simulink model "induction_motor_load_step"  (R2021a)
settings: Solver=VariableStepAuto  StartTime=0.0  StopTime=3  FixedStep=0.000001  MaxStep=0.000001  MinStep=0.0000001  RelTol=1e-7
values from neighbouring files (symbols this model uses):
  A1 = [-1/(ts*sig) 0 lm/(ls*tr*sig) 0;0 -1/(ts*sig) 0 lm/(ls*tr*sig);lm/(lr*ts*sig) 0 -1/(tr*sig) 0; 0 lm/(lr*ts*sig) 0 -1/(tr*sig)]    [induction_motor_parameters.m]
  A2 = [0 1 0 0; -1 0 0 0;0 0 0 1;0 0 -1 0]    [induction_motor_parameters.m]
  A3 = [0 1/sig 0 lm/(ls*sig);-1/sig 0 -lm/(ls*sig) 0;0 -lm/(lr*sig) 0 -lm*lm/(ls*lr*sig); lm/(lr*sig) 0 lm*lm/(ls*lr*sig) 0]    [induction_motor_parameters.m]
  B = [1/(ls*sig) 0 0 0;0 1/(ls*sig) 0 0; -lm/(ls*lr*sig) 0 0 0;0 -lm/(ls*lr*sig) 0 0 ]    [induction_motor_parameters.m]
  fr = 0.0015    [induction_motor_parameters.m]
  j = 0.0056    [induction_motor_parameters.m]
  L = [ls 0 lm 0;0 ls 0 lm;lm 0 lr 0;0 lm 0 lr]    [induction_motor_parameters.m]
  lm = 0.069    [induction_motor_parameters.m]
  lr = 0.071    [induction_motor_parameters.m]
  p = 2    [induction_motor_parameters.m]
  T = [2/3 -1/3 -1/3 ; -1/3 2/3 -1/3;-1/3 -1/3 2/3]    [induction_motor_parameters.m]
  T_dent = t/m    (= 0.000952380952381)    [induction_motor_parameters.m]
libraries: spsabctodq0Lib x1, spsdq0toabcLib x1, simulink x1, spspowerguiLib x1

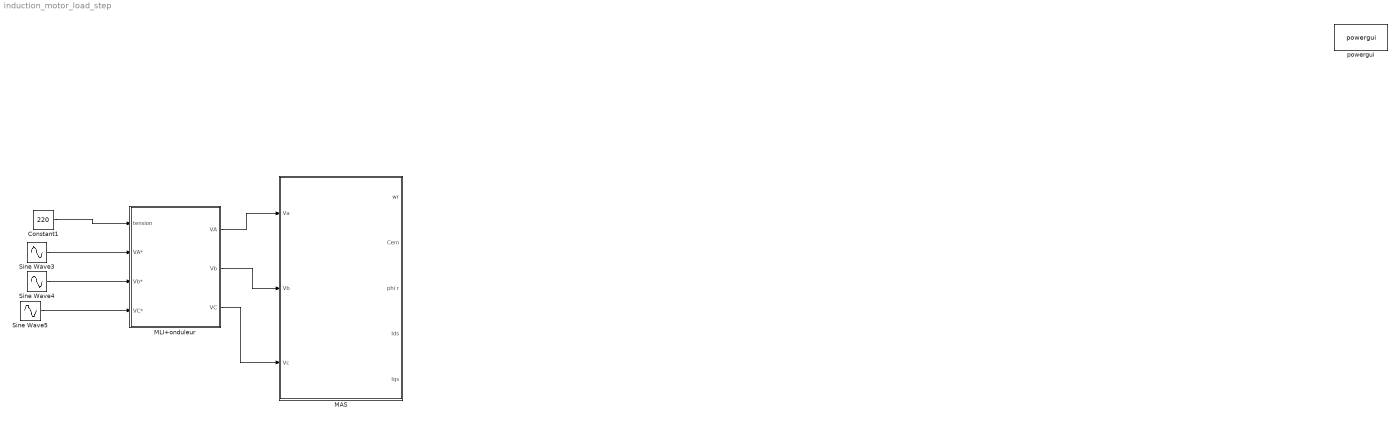
== system induction_motor_load_step ==
  Constant1 : Constant  Value=220
  "MAS " : Subsystem
  MLI+onduleur : Subsystem
  Sine Wave3 : Sin  Amplitude=220  Frequency=2*pi*50  SampleTime=0
  Sine Wave4 : Sin  Amplitude=220  Frequency=2*pi*50  Phase=-2*pi/3  SampleTime=0
  Sine Wave5 : Sin  Amplitude=220  Frequency=2*pi*50  Phase=-4*pi/3  SampleTime=0
  powergui : spspowerguiLib/powergui  Priority=1  SimulationMode=Discrete  SampleTime=50e-7  frequency=60  Iterations=50  frequencyindice=0  Pbase=100e6  ErrMax=1e-4  UnitsV=kV  UnitsW=MW  buscounter=0  FunctionMessages=off  echomessages=off  EnableUseOfTLC=off  CurrentSourceSwitches=off  DisableSnubberDevices=off  DisableRonSwitches=off  DisableVfSwitches=off  DisplayEquations=off  AutomaticDiscreteSolvers=off  SolverType=Tustin/Backward Euler (TBE)  Interpol=off  ExternalGateDelay=off  methode=off  Ts=100  x0status=blocks  SPID=on  SwTol=0  HookPort=off  NonlinearTolerance=1e-4  nMaxIteration=100  ContinueOnMaxIteration=off  RestoreLinks=warning  ResistiveCurrentMeasurement=off  Frange=[0:2:500]  Ylog=off  Xlog=on  ShowGrid=off  save=off  variable=ZData  structure=0  ZoomFFT=off  StartTime=0.0  cycles=1  DisplayStyle=1  fundamental=60  FreqAxis=off  MaxFrequency=1000  frequencyindicesteady=1  RmsSteady=1  display=off
  wires:
  MLI+onduleur/2(Vb) -> "MAS "/2(Vb)
  MLI+onduleur/3(VC) -> "MAS "/3(Vc)
  MLI+onduleur/1(VA) -> "MAS "/1(Va)
  Sine Wave3/1 -> MLI+onduleur/2(VA*)
  Sine Wave5/1 -> MLI+onduleur/4(VC*)
  Sine Wave4/1 -> MLI+onduleur/3(Vb*)
  Constant1/1 -> MLI+onduleur/1(tension)

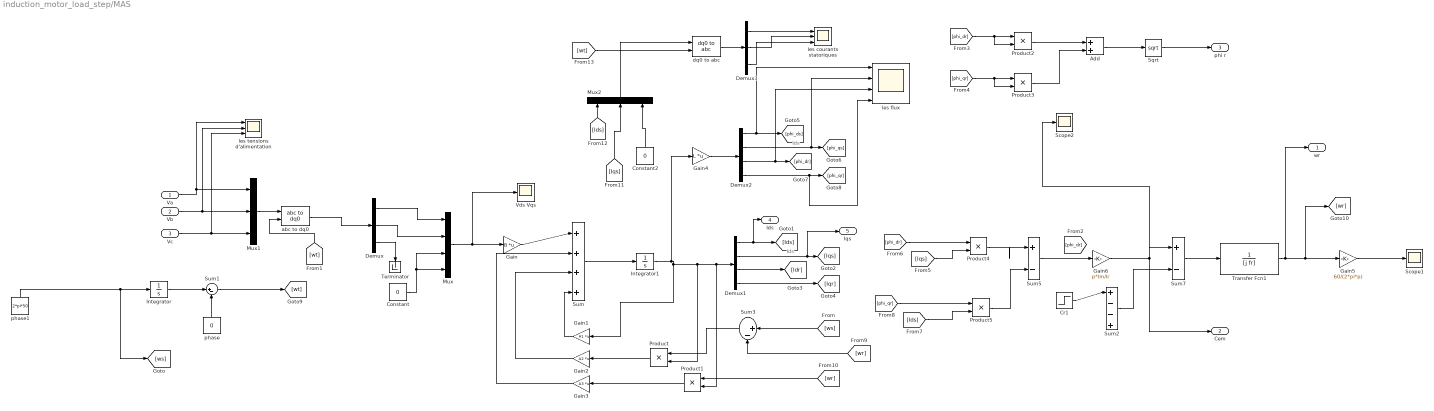
== system induction_motor_load_step/MAS  ==
  note: Ids
  note: Ids
  Va : Inport
  Vb : Inport  Port=2
  Vc : Inport  Port=3
  Add : Sum
  Constant : Constant  Value=0
  Constant2 : Constant  Value=0
  Cr1 : Step  After=10  SampleTime=0
  Demux : Demux  Outputs=3
  Demux1 : Demux
  Demux2 : Demux
  Demux3 : Demux  Outputs=3
  Gain : Gain  Gain=B  Multiplication=Matrix(K*u)
  Gain1 : Gain  Gain=A1  Multiplication=Matrix(K*u)
  Gain2 : Gain  Gain=A2  Multiplication=Matrix(K*u)
  Gain3 : Gain  Gain=A3  Multiplication=Matrix(K*u)
  Gain4 : Gain  Gain=L  Multiplication=Matrix(K*u)
  Gain5 : Gain  Gain=60/(2*pi*p)
  Gain6 : Gain  Gain=p*lm/lr
  Integrator : Integrator
  Integrator1 : Integrator
  Mux : Mux
  Mux1 : Mux  Inputs=3
  Mux2 : Mux  Inputs=3
  Product{,1..5} (6 alike) : Product
  Scope1 : Scope
  Scope2 : Scope
  Sqrt : Sqrt  SaturateOnIntegerOverflow=on
  Sum : Sum  Inputs=|++++
  Sum{1,3,5,7} (4 alike) : Sum  Inputs=|+-
  Sum2 : Sum  Inputs=|+--+
  Terminator : Terminator
  Transfer Fcn1 : TransferFcn  Denominator=[j fr]
  Vds Vqs : Scope
  abc to dq0 : spsabctodq0Lib/abc to dq0  Alignment=Aligned with phase A axis
  dq0 to abc : spsdq0toabcLib/dq0 to abc  Alignment=90 degrees behind phase A axis
  les courants statoriques : Scope  NumInputPorts=3
  les flux : Scope  NumInputPorts=4
  "les tensions d'alimentation " : Scope  NumInputPorts=3
  phase : Constant  Value=0
  phase1 : Constant  Value=2*pi*50
  wr : Outport
  Cem : Outport  Port=2
  phi r : Outport  Port=3
  Ids : Outport  Port=4
  Iqs : Outport  Port=5
  wires:
  Product/1 -> Gain2/1
  [wr] -> Product1/1
  Transfer Fcn1/1 -> wr/1, Gain5/1, [wr]
  Demux2/1 -> les flux/1, [phi_ds]
  Gain2/1 -> Sum/3
  Gain/1 -> Sum/1
  Constant2/1 -> Mux2/3
  Sum3/1 -> Product/1
  [Iqs] -> Product4/2
  Gain4/1 -> Demux2/1
  Demux2/3 -> les flux/3, [phi_dr]
  [wt] -> dq0 to abc/2
  Constant/1 -> Mux/4, Mux/3
  [phi_dr] -> Product4/1
  phase/1 -> Sum1/2
  Integrator1/1 -> Gain4/1, Product/2, Product1/2, Demux1/1, Gain1/1
  Demux/3 -> Terminator/1
  Demux/2 -> Mux/2
  [ws] -> Sum3/1
  Demux2/2 -> les flux/2, [phi_qs]
  Integrator/1 -> Sum1/1
  Demux1/4 -> [Iqr]
  Demux1/3 -> [Idr]
  Demux1/1 -> Ids/1, [Ids]
  Sum1/1 -> [wt]
  Gain3/1 -> Sum/2
  Mux/1 -> Vds Vqs/1, Gain/1
  Gain6/1 -> Cem/1, Scope2/1, Sum7/1
  Product1/1 -> Gain3/1
  Mux2/1 -> dq0 to abc/1
  Gain1/1 -> Sum/4
  [wr] -> Sum3/2
  Sum7/1 -> Transfer Fcn1/1
  Sum5/1 -> Gain6/1
  [Ids] -> Product5/2
  [phi_qr] -> Product5/1
  Demux1/2 -> Iqs/1, [Iqs]
  Demux/1 -> Mux/1
  Sum/1 -> Integrator1/1
  Product4/1 -> Sum5/1
  Product5/1 -> Sum5/2
  [Iqs] -> Mux2/2
  [Ids] -> Mux2/1
  phase1/1 -> Integrator/1, [ws]
  Va/1 -> "les tensions d'alimentation "/1, Mux1/1
  Vc/1 -> "les tensions d'alimentation "/3, Mux1/3
  Mux1/1 -> abc to dq0/1
  [wt] -> abc to dq0/2
  abc to dq0/1 -> Demux/1
  [phi_dr] -> Product2/2, Product2/1
  [phi_qr] -> Product3/2, Product3/1
  Product2/1 -> Add/1
  Product3/1 -> Add/2
  Add/1 -> Sqrt/1
  Sqrt/1 -> phi r/1
  Demux2/4 -> les flux/4, [phi_qr]
  dq0 to abc/1 -> Demux3/1
  Demux3/1 -> les courants statoriques/1
  Demux3/2 -> les courants statoriques/2
  Demux3/3 -> les courants statoriques/3
  Sum2/1 -> Sum7/2
  Vb/1 -> "les tensions d'alimentation "/2, Mux1/2
  Gain5/1 -> Scope1/1
  Cr1/1 -> Sum2/1

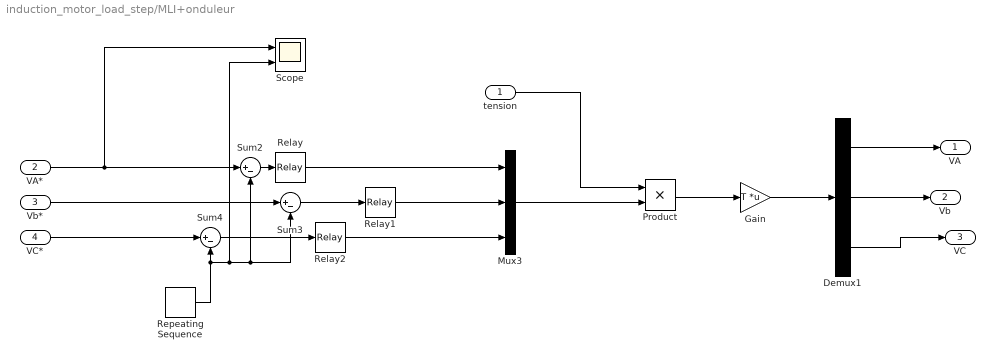
== system induction_motor_load_step/MLI+onduleur ==
  tension : Inport
  VA* : Inport  Port=2
  Vb* : Inport  Port=3
  VC* : Inport  Port=4
  Demux1 : Demux  Outputs=3
  Gain : Gain  Gain=T  Multiplication=Matrix(K*u)
  Mux3 : Mux  Inputs=3
  Product : Product
  Relay : Relay  OffOutputValue=-1
  Relay1 : Relay  OffOutputValue=-1
  Relay2 : Relay  OffOutputValue=-1
  Repeating Sequence : simulink/Sources/Repeating Sequence  rep_seq_t="[0  T_dent/2 T_dent ]"  rep_seq_y=[-350 350 -350]
  Scope : Scope  NumInputPorts=2
  Sum2 : Sum  Inputs=|+-
  Sum3 : Sum  Inputs=|+-
  Sum4 : Sum  Inputs=|+-
  VA : Outport
  Vb : Outport  Port=2
  VC : Outport  Port=3
  wires:
  Relay/1 -> Mux3/1
  Repeating Sequence/1 -> Scope/2, Sum2/2, Sum3/2, Sum4/2
  Product/1 -> Gain/1
  Relay1/1 -> Mux3/2
  Sum3/1 -> Relay1/1
  Mux3/1 -> Product/2
  Relay2/1 -> Mux3/3
  Sum2/1 -> Relay/1
  Sum4/1 -> Relay2/1
  Gain/1 -> Demux1/1
  tension/1 -> Product/1
  Vb*/1 -> Sum3/1
  Demux1/2 -> Vb/1
  VC*/1 -> Sum4/1
  VA*/1 -> Scope/1, Sum2/1
  Demux1/3 -> VC/1
  Demux1/1 -> VA/1
